simulink model "relay_feedback.slx"  (R2024b)
settings: Solver=VariableStepAuto  StartTime=0.0  StopTime=50  RelTol=1e-3
settings Model: Creator=bashi  LastModifiedBy=bashi

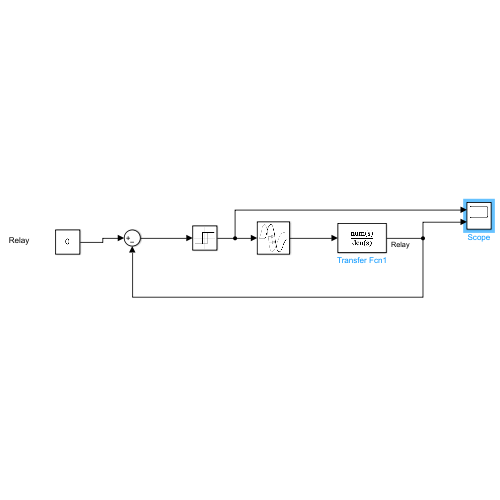
[thumbnail: Simulink's stored preview of the top-level diagram]
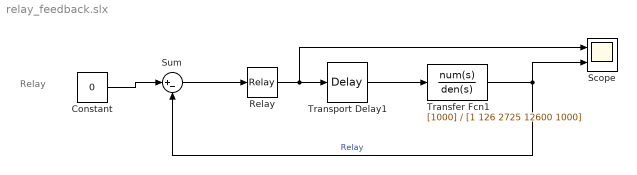
== system relay_feedback.slx ==
  note: Relay
  Constant : Constant  Value=0
  Relay : Relay  OnSwitchValue=0  OffSwitchValue=0  OffOutputValue=-1
  Scope : Scope  NumInputPorts=2
  Sum : Sum  Inputs=|+-
  Transfer Fcn1 : TransferFcn  Numerator=[1000]  Denominator=[1 126 2725 12600 1000]
  Transport Delay1 : TransportDelay  DelayTime=2.5
  wires:
  Sum/1 -> Relay/1
  Transfer Fcn1/1 -> Sum/2, Scope/2  "Relay"
  Relay/1 -> Scope/1, Transport Delay1/1
  Transport Delay1/1 -> Transfer Fcn1/1
  Constant/1 -> Sum/1
